simulink model "Zero_Perturb_MPPT_Live"  (R2025a)
settings: Solver=ode23t  StopTime=2  FixedStep=1e-6  MaxStep=2e-6
InitFcn:
  | if ~exist('PI_Preset','var'), PI_Preset = 'sun'; end
  | switch PI_Preset
  |   case 'bench'  % doc constants, indoor-lamp bench (3-5% duty)
  |     PI_Kp=1.2; PI_Ki=0.5; PI_Vdb=0.04; PI_Umax=600; PI_Slew=1; PI_Duty0=150;
  |   otherwise       % full-sun / cloud transient (retuned, see report)
  |     PI_Kp=100; PI_Ki=2500; PI_Vdb=0.04; PI_Umax=3900; PI_Slew=1000; PI_Duty0=2500;
  | end
  | PI_Ts = 0.05;
StartFcn:
  | fprintf('\n[SIMULINK LIVE] Simulation Started. Streaming to http://localhost:3000...\n');
StopFcn:
  | fprintf('\n[SIMULINK LIVE] Simulation Stopped.\n');
libraries: nesl_utility x6, fl_lib x5, ee_lib x3, simulink x1
(part 1 of 2)
settings Model: Creator=admin  LastModifiedBy=saisi
settings SolverCC: ZeroCrossAlgorithm=Adaptive
settings DebuggingCC: AlgebraicLoopMsg=none

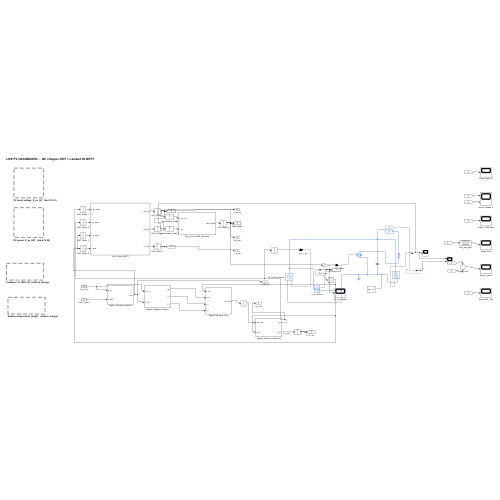
[thumbnail: Simulink's stored preview of the top-level diagram]
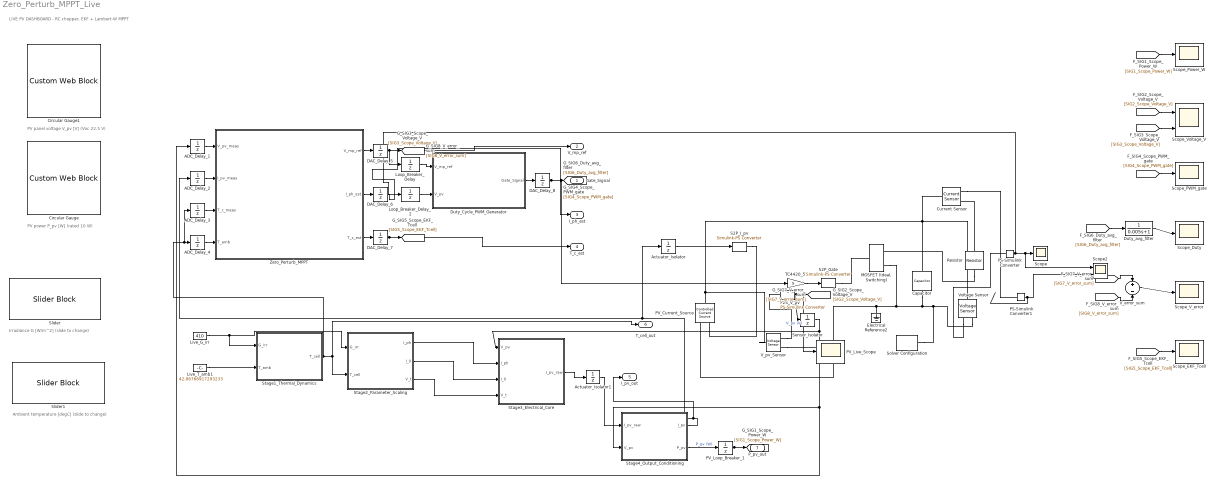
== system Zero_Perturb_MPPT_Live ==
  note: LIVE PV DASHBOARD - RC chopper, EKF + Lambert-W MPPT
  note: PV panel voltage V_pv [V] (Voc 22.5 V)
  note: PV power P_pv [W] (rated 10 W)
  note: Irradiance G [W/m^2] (slide to change)
  note: Ambient temperature [degC] (slide to change)
  ADC_Delay_{1..4} (4 alike) : UnitDelay  SampleTime=-1
  Actuator_Isolator : UnitDelay  SampleTime=-1
  Actuator_Isolator1 : UnitDelay  SampleTime=-1
  Capacitor : ee_lib/Passive/Capacitor  cap_option=ee.enum.passive.capacitor.capOption.const  c=470e-6 F  Cvec=[1e-05, 1e-06] F  Vvec=[0, 10] V  CV_table_symmetry=ee.enum.passive.capacitor.tableSymmetry.yes  f_vec=[1, 10] kHz  DFext_vec=[.8, 1.2]  enable_C_tol=ee.enum.toleranceApplication.none  averaging_period=0 s  C_tol=5  tol_distribution=ee.enum.toleranceDistribution.uniform  nSigma=4  r=0 Ohm  g=0 1/Ohm  enable_operating_limits=ee.enum.enable.no  operating_limit_action=ee.enum.passive.reportOpLim.warn  max_working_voltage_range=[-25, 25] V  power_rating=1 W  maxTemperature=85 degC  thermalEnable=false  thermalMass=1 J/K  i_specify=off  i_priority=None  i=0 A  i_nominal_specify=off  i_nominal_value=1  i_nominal_unit=A  v_specify=off  v_priority=None  v=0 V  v_nominal_specify=off  v_nominal_value=1  v_nominal_unit=V  vc_specify=off  vc_priority=High  vc=0 V  vc_nominal_specify=off  vc_nominal_value=1  vc_nominal_unit=V  T_specify=off  T_priority=None  T=298.15 K  T_nominal_specify=off  T_nominal_value=1  T_nominal_unit=K
  Circular Gauge : CustomWebBlock  ShowInitialText=on  Configuration="{\"components\":[{\"name\":\"CircularScaleComponent\",\"settings\":{\"bounds\":{\"max\":15,\"min\":0,\"tickInterval\":\"auto\"},\"direction\":\"cw\",\"flipLimits\":0,\"innerRadius\":0.75,\"internalTickHeightScaleFactor\":1,\"labelColor\":[255,255,200],\"labelFont\":{\"font\":\"Arial\",\"fontSize\":12},\"labelRadius\":0.528,\"labelTransparency\":1,\"minorTickHeightScaleFactor\":0.2,\"needleImage\":{\"size\":[200,50],\"src\":\"data:image\\/svg+xml;base64,PD94bWwgdmVyc2lvbj0iMS4wIiBlbmNvZGluZz0idXRmLTgiPz4KPCEtLSBHZW5lcmF0b3I6IEFkb2JlIElsbHVzdHJhdG9yIDI0LjEuMiwgU1ZHIEV4cG9ydCBQbHVnLUluIC4gU1ZHIFZlcnNpb246IDYuMDAgQnVpbGQgMCkgIC0tPgo8c3ZnIHZlcnNpb249IjEuMSIgaWQ9IkxheWVyXzEiIHhtbG5zPSJodHRwOi8vd3d3LnczLm9yZy8yMDAwL3N2ZyIgeG1sbnM6eGxpbms9Imh0dHA6Ly93d3cudzMub3JnLzE5OTkveGxpbmsiIHg9IjBweCIgeT0iMHB4IgoJIHZpZXdCb3g9IjAgMCAyMDAgNTAiIHN0eWxlPSJlbmFibGUtYmFja2dyb3VuZDpuZXcgMCAwIDIwMCA1MDsiIHhtbDpzcGFjZT0icHJlc2VydmUiPgo8c3R5bGUgdHlwZT0idGV4dC9jc3MiPgoJLnN0MHtmaWxsOiNFQzIxMjc7fQo8L3N0eWxlPgo8cGF0aCBjbGFzcz0ic3QwIiBkPSJNMTYyLjgsMTMuN0MxNjksNC40LDE4MS43LDEuOSwxOTEsOC4xczExLjgsMTguOSw1LjYsMjguMnMtMTguOSwxMS44LTI4LjIsNS42bDAsMAoJQzE1OS4xLDM1LjYsMTU2LjYsMjMsMTYyLjgsMTMuN0wxNjIuOCwxMy43eiBNMTY1LjgsMTUuOGMtNS4xLDcuNi0zLjEsMTcuOSw0LjYsMjNjNy42LDUuMSwxNy45LDMuMSwyMy00LjYKCWM1LjEtNy42LDMuMS0xNy45LTQuNi0yM2wwLDBDMTgxLjIsNi4yLDE3MC45LDguMiwxNjUuOCwxNS44eiIvPgo8cGF0aCBjbGFzcz0ic3QwIiBkPSJNMC40LDI1Ljl2LTMuM2wxNTktMi41Yy0wLjcsMi42LTAuNyw1LjIsMCw3LjhMMC40LDI1Ljl6Ii8+CjxjaXJjbGUgY2xhc3M9InN0MCIgY3g9IjE3OS42IiBjeT0iMjQiIHI9IjAuNyIvPgo8L3N2Zz4K\"},\"needleOffset\":[0.18464878250906522,0],\"needleOrientation\":-45,\"needleRotation\":180,\"needleSize\":{\"height\":0.11741692305346914,\"width\":0.46108337545091255},\"outerRadius\":0.9,\"position\":[0.05,0.05,0.9,0.9],\"referencePoint\":\"auto\",\"scaleAngle\":270,\"scaleAngleOffset\":135,\"scaleColors\":[],\"scaleColorsSize\":0.2,\"scaleDirection\":\"CW\",\"scalePosition\":[0,0,1,1],\"showLabels\":1,\"showMinorTicks\":1,\"showSpanLine\":1,\"showTicks\":1,\"tickColor\":[252,252,197],\"tickTransparency\":1,\"valueBarColor\":[0,114,189],\"valueBarPosition\":[0,0,1,1],\"valueBarSize\":0.2,\"valueBarTransparency\":1}},{\"name\":\"BackgroundImageComponent\",\"settings\":{\"image\":{\"size\":[500,500],\"src\":\"data:image\\/svg+xml;base64,PD94bWwgdmVyc2lvbj0iMS4wIiBlbmNvZGluZz0iVVRGLTgiIHN0YW5kYWxvbmU9Im5vIj8+CjxzdmcKICAgeG1sbnM6ZGM9Imh0dHA6Ly9wdXJsLm9yZy9kYy9lbGVtZW50cy8xLjEvIgogICB4bWxuczpjYz0iaHR0cDovL2NyZWF0aXZlY29tbW9ucy5vcmcvbnMjIgogICB4bWxuczpyZGY9Imh0dHA6Ly93d3cudzMub3JnLzE5OTkvMDIvMjItcmRmLXN5bnRheC1ucyMiCiAgIHhtbG5zOnN2Zz0iaHR0cDovL3d3dy53My5vcmcvMjAwMC9zdmciCiAgIHhtbG5zPSJodHRwOi8vd3d3LnczLm9yZy8yMDAwL3N2ZyIKICAgeG1sbnM6 ...(+9964 chars)\"},\"position\":[0,0,1,1],\"scaleMode\":\"0\"}},{\"name\":\"ForegroundImageComponent\",\"settings\":{\"image\":{\"size\":[0,0],\"src\":\"default\",\"srcOrientation\":[]},\"isForeground\":1,\"position\":[0,0,1,1],\"scaleMode\":\"0\"}}],\"derived\":{\"blockParameters\":{\"ForegroundColor\":[0.9882352941176471,0.9882352941176471,0.7725490196078432],\"Limits\":{\"Max\":15,\"Min\":0,\"Ticks\":\"auto\"},\"ScaleColors\":[],\"ScaleDirection\":\"Clockwise\",\"ScaleMax\":15,\"ScaleMin\":0,\"TickInterval\":\"auto\",\"fixedAspectRatio\":\"on\"}},\"settings\":{\"BindingType\":\"signal\",\"aspectRatio\":1.032258064516129,\"backgroundColor\":[0,0,0,\"1\"],\"backgroundOffset\":1,\"backgroundOpacity\":1,\"direction\":\"cw\",\"fixedAspectRatio\":\"on\",\"flipLimits\":0,\"orientation\":\"horizontal\",\"showBackgroundColor\":false,\"value\":0,\"version\":\"R2023a\"},\"type\":\"CircularGauge\"}"
  Circular Gauge1 : CustomWebBlock  ShowInitialText=on  Configuration="{\"components\":[{\"name\":\"CircularScaleComponent\",\"settings\":{\"bounds\":{\"max\":25,\"min\":0,\"tickInterval\":\"auto\"},\"direction\":\"cw\",\"flipLimits\":0,\"innerRadius\":0.75,\"internalTickHeightScaleFactor\":1,\"labelColor\":[255,255,200],\"labelFont\":{\"font\":\"Arial\",\"fontSize\":12},\"labelRadius\":0.528,\"labelTransparency\":1,\"minorTickHeightScaleFactor\":0.2,\"needleImage\":{\"size\":[200,50],\"src\":\"data:image\\/svg+xml;base64,PD94bWwgdmVyc2lvbj0iMS4wIiBlbmNvZGluZz0idXRmLTgiPz4KPCEtLSBHZW5lcmF0b3I6IEFkb2JlIElsbHVzdHJhdG9yIDI0LjEuMiwgU1ZHIEV4cG9ydCBQbHVnLUluIC4gU1ZHIFZlcnNpb246IDYuMDAgQnVpbGQgMCkgIC0tPgo8c3ZnIHZlcnNpb249IjEuMSIgaWQ9IkxheWVyXzEiIHhtbG5zPSJodHRwOi8vd3d3LnczLm9yZy8yMDAwL3N2ZyIgeG1sbnM6eGxpbms9Imh0dHA6Ly93d3cudzMub3JnLzE5OTkveGxpbmsiIHg9IjBweCIgeT0iMHB4IgoJIHZpZXdCb3g9IjAgMCAyMDAgNTAiIHN0eWxlPSJlbmFibGUtYmFja2dyb3VuZDpuZXcgMCAwIDIwMCA1MDsiIHhtbDpzcGFjZT0icHJlc2VydmUiPgo8c3R5bGUgdHlwZT0idGV4dC9jc3MiPgoJLnN0MHtmaWxsOiNFQzIxMjc7fQo8L3N0eWxlPgo8cGF0aCBjbGFzcz0ic3QwIiBkPSJNMTYyLjgsMTMuN0MxNjksNC40LDE4MS43LDEuOSwxOTEsOC4xczExLjgsMTguOSw1LjYsMjguMnMtMTguOSwxMS44LTI4LjIsNS42bDAsMAoJQzE1OS4xLDM1LjYsMTU2LjYsMjMsMTYyLjgsMTMuN0wxNjIuOCwxMy43eiBNMTY1LjgsMTUuOGMtNS4xLDcuNi0zLjEsMTcuOSw0LjYsMjNjNy42LDUuMSwxNy45LDMuMSwyMy00LjYKCWM1LjEtNy42LDMuMS0xNy45LTQuNi0yM2wwLDBDMTgxLjIsNi4yLDE3MC45LDguMiwxNjUuOCwxNS44eiIvPgo8cGF0aCBjbGFzcz0ic3QwIiBkPSJNMC40LDI1Ljl2LTMuM2wxNTktMi41Yy0wLjcsMi42LTAuNyw1LjIsMCw3LjhMMC40LDI1Ljl6Ii8+CjxjaXJjbGUgY2xhc3M9InN0MCIgY3g9IjE3OS42IiBjeT0iMjQiIHI9IjAuNyIvPgo8L3N2Zz4K\"},\"needleOffset\":[0.18464878250906522,0],\"needleOrientation\":-45,\"needleRotation\":180,\"needleSize\":{\"height\":0.11741692305346914,\"width\":0.46108337545091255},\"outerRadius\":0.9,\"position\":[0.05,0.05,0.9,0.9],\"referencePoint\":\"auto\",\"scaleAngle\":270,\"scaleAngleOffset\":135,\"scaleColors\":[],\"scaleColorsSize\":0.2,\"scaleDirection\":\"CW\",\"scalePosition\":[0,0,1,1],\"showLabels\":1,\"showMinorTicks\":1,\"showSpanLine\":1,\"showTicks\":1,\"tickColor\":[252,252,197],\"tickTransparency\":1,\"valueBarColor\":[0,114,189],\"valueBarPosition\":[0,0,1,1],\"valueBarSize\":0.2,\"valueBarTransparency\":1}},{\"name\":\"BackgroundImageComponent\",\"settings\":{\"image\":{\"size\":[500,500],\"src\":\"data:image\\/svg+xml;base64,PD94bWwgdmVyc2lvbj0iMS4wIiBlbmNvZGluZz0iVVRGLTgiIHN0YW5kYWxvbmU9Im5vIj8+CjxzdmcKICAgeG1sbnM6ZGM9Imh0dHA6Ly9wdXJsLm9yZy9kYy9lbGVtZW50cy8xLjEvIgogICB4bWxuczpjYz0iaHR0cDovL2NyZWF0aXZlY29tbW9ucy5vcmcvbnMjIgogICB4bWxuczpyZGY9Imh0dHA6Ly93d3cudzMub3JnLzE5OTkvMDIvMjItcmRmLXN5bnRheC1ucyMiCiAgIHhtbG5zOnN2Zz0iaHR0cDovL3d3dy53My5vcmcvMjAwMC9zdmciCiAgIHhtbG5zPSJodHRwOi8vd3d3LnczLm9yZy8yMDAwL3N2ZyIKICAgeG1sbnM6 ...(+9964 chars)\"},\"position\":[0,0,1,1],\"scaleMode\":\"0\"}},{\"name\":\"ForegroundImageComponent\",\"settings\":{\"image\":{\"size\":[0,0],\"src\":\"default\",\"srcOrientation\":[]},\"isForeground\":1,\"position\":[0,0,1,1],\"scaleMode\":\"0\"}}],\"derived\":{\"blockParameters\":{\"ForegroundColor\":[0.9882352941176471,0.9882352941176471,0.7725490196078432],\"Limits\":{\"Max\":25,\"Min\":0,\"Ticks\":\"auto\"},\"ScaleColors\":[],\"ScaleDirection\":\"Clockwise\",\"ScaleMax\":25,\"ScaleMin\":0,\"TickInterval\":\"auto\",\"fixedAspectRatio\":\"on\"}},\"settings\":{\"BindingType\":\"signal\",\"aspectRatio\":1.032258064516129,\"backgroundColor\":[0,0,0,\"1\"],\"backgroundOffset\":1,\"backgroundOpacity\":1,\"direction\":\"cw\",\"fixedAspectRatio\":\"on\",\"flipLimits\":0,\"orientation\":\"horizontal\",\"showBackgroundColor\":false,\"value\":0,\"version\":\"R2023a\"},\"type\":\"CircularGauge\"}"
  Current Sensor : fl_lib/Electrical/Electrical Sensors/Current Sensor
  DAC_Delay_{5..8} (4 alike) : UnitDelay  SampleTime=-1
  Duty_Cycle_PWM_Generator : Subsystem
  Duty_avg_filter : TransferFcn  Numerator=1  Denominator=[0.005 1]
  Electrical Reference2 : fl_lib/Electrical/Electrical Elements/Electrical Reference
  Live_G_irr : Constant  Value=410
  Live_T_amb1 : Constant  Value=42.06766917293233
  Loop_Breaker_Delay : UnitDelay  SampleTime=-1
  Loop_Breaker_Delay_2 : UnitDelay  SampleTime=-1
  "MOSFET (Ideal, Switching)" : ee_lib/Semiconductors & Converters/MOSFET (Ideal, Switching)  port_option=ee.enum.controlport.ps  Rds=0.022 Ohm  Goff=1e-6 1/Ohm  Vth=1.5 V  diode_param=ee.enum.semiconductors.protectionDiode.nodynamics  diode_Vf=0.8 V  diode_Ron=0.001 Ohm  diode_Goff=1e-5 1/Ohm  diode_C=50e-9 F  diode_iRM=-235 A  diode_iF=300 A  diode_idot=-50 A/us  diode_trr_param=ee.enum.converters.diodeReverseParam.trr_factor  diode_trr_factor=3  diode_trr=15 us  diode_Qrr=1500 s*uA  ids_specify=off  ids_priority=None  ids=0 A  ids_nominal_specify=off  ids_nominal_value=1  ids_nominal_unit=A  vds_specify=off  vds_priority=None  vds=0 V  vds_nominal_specify=off  vds_nominal_value=1  vds_nominal_unit=V  vgs_specify=off  vgs_priority=None  vgs=0 V  vgs_nominal_specify=off  vgs_nominal_value=1  vgs_nominal_unit=V  thermal_loss_option=ee.enum.converters.thermalLossOption.constantvalues  Von_data=[0, 1.8, 3.2, 6, 10, 16; 0, 2, 5.5, 9.5, 15, 25] V  Tj=[298.15, 448.15] K  Iout_data=[0, 20, 40, 60, 80, 100] A  tabulateWithVds=false  Eon_data=[0, 55.04, 124.57, 235.53, 362.12; 0, 71.25, 161.25, 304.88, 468.75] * 1e-6 J  Eoff_data=[0, 18, 30, 56.1, 76.5; 0, 22.5, 37.5, 70.13, 95.63] * 1e-6 J  Eon_data_3D=[zeros(2, 5, 3)] J  Eoff_data_3D=[zeros(2, 5, 3)] J  Tj_loss=[298.15, 448.15] K  Iout_data_loss=[0, 10, 20, 30, 40] A  Vds_loss=[0, 150, 300] V  Eon_scalar=22.86e-3 J  Eoff_scalar=17.14e-3 J  Voff=300 V  Iout_scalar=600 A  useCurrentFromPreviousCycle=false  useVoltageFromPreviousCycle=false  diodeModelType=ee.enum.converters.diodeModelType.pwl  diodeTableType=ee.enum.diode.tableType.IfMat  diode_ReverseIVType=ee.enum.diode.diodeReverseIV.constant  diode_IfMat=[.07, .12, .19, 1.75, 4.24, 7.32, 11.2; .16, .3, .72, 2.14, 4.02, 6.35, 9.12] A  diode_VfMat=[.9, 1.15, 1.25, 1.5, 1.75, 2.17, 2.6, 2.85; .58, .68, .75, 1.1, 1.38, 1.77, 2.27, 2.7] V  diode_TjVec=[25, 125] degC  diode_VfVec=[.5, .7, .9, 1.3, 1.7, 2.1, 2.5] V  diode_IfVec=[.1, .2, .5, 1, 2, 4, 7, 10] A  diode_IrMat=[1e-06, 2e-06, 5e-06, 1e-05, 2.5e-05, 5e-05, .0001; 2e-06, 5e-06, 1e-05, 4e-05, 8e-05, .0002, .0005] A  diode_VrMat=[10, 100, 200, 250, 300, 325, 350; 10, 70, 160, 220, 270, 300, 320] V  diode_VrVec=[10, 20, 40, 50, 70, 80, 100] V  diode_IrVec=[1e-06, 2e-06, 5e-06, 1e-05, 2e-05, 5e-05, .0001] A  diode_Vr=-600 V  diode_Ls=150 nH  diode_Erec=0.03 J  diode_rec_loss_model=ee.enum.diode.reverseRecoveryModelTabulateUpTo3D.fixed  diode_ErecVal=0 J  diode_scaleWithIandV=true  diode_ErecMat=zeros(2, 3) J  diodeErecMat3D=zeros(2, 3, 2) J  diode_TjrecVec=[298.15, 398.15] K  diode_IfrecVec=[.1, 1, 10] A  diodeVrecVec=[0, 100] V  diode_IrecVal=10 A  diode_VrecVal=10 V  diode_tFilter=1 / 1000 / 100 s  separateThermalPortForDiode=false  thermal_network_parameterization=ee.enum.thermalNetworkTopology.external  Rth=[.03, .2] K/W  Rth_Cauer=[.03, .1, .2] K/W  Rth_Foster=[.08, .14, .22, .16] K/W  thermal_mass_parameterization=ee.enum.thermalNetwork.timeconstant  thermal_mass=[3, 25] J/K  thermal_mass_Cauer=[3, 10, 25] J/K  thermal_mass_Foster=[.001, .005, .05, .5] J/K  thermal_time_constant=[.1, 5] s  thermal_time_constant_Cauer=[.1, 1, 5] s  thermal_time_constant_Foster=[7e-05, .0007, .01, .08] s  thermal_mass_initial_temperatures=[25, 25] degC  thermal_mass_initial_temperatures_Cauer=[25, 25, 25] degC  junction_thermal_mass=0.1 J/K  Tvec_initial_Foster=[25, 25, 25, 25] degC  RthDiode=[.03, .2] K/W  RthCauerDiode=[.03, .1, .2] K/W  RthFosterDiode=[.03, .2] K/W  thermalMassDiode=[3, 25] J/K  thermalMassCauerDiode=[3, 10, 25] J/K  thermalMassFosterDiode=[33, 50] J/K  thermalTauDiode=[.1, 5] s  thermalTauCauerDiode=[.1, 1, 5] s  thermalTauFosterDiode=[1, 10] s  thermalMassInitTempDiode=[25, 25] degC  thermalMassInitTempCauerDiode=[25, 25, 25] degC  junctionthermalMassDiode=0.1 J/K  TVecInitialFosterDiode=[25, 25, 25, 25] degC  no_thermal_network=ee.enum.enable.no  mosfet_junction_temperature_specify=off  mosfet_junction_temperature_priority=None  mosfet_junction_temperature=25 degC  mosfet_junction_temperature_nominal_specify=off  mosfet_junction_temperature_nominal_value=1  mosfet_junction_temperature_nominal_unit=degC  diode_junction_temperature_specify=off  diode_junction_temperature_priority=None  diode_junction_temperature=25 degC  diode_junction_temperature_nominal_specify=off  diode_junction_temperature_nominal_value=1  diode_junction_temperature_nominal_unit=degC  Qj_specify=off  Qj_priority=None  Qj=0 W  Qj_nominal_specify=off  Qj_nominal_value=1  Qj_nominal_unit=W  accumulatedSwitchingLosses_specify=off  accumulatedSwitchingLosses_priority=None  accumulatedSwitchingLosses=0 J
  P2S_V_pv : nesl_utility/PS-Simulink Converter  PhysicalDomain=network_engine_domain  SubClassName=ps_output  LeftPortType=input  RightPortType=output  PseudoPeriodic=off  Frequencies=[]  VectorFormat=inherit  Unit=inherit  AffineConversion=off
  PS-Simulink Converter : nesl_utility/PS-Simulink Converter  PhysicalDomain=network_engine_domain  SubClassName=ps_output  LeftPortType=input  RightPortType=output  PseudoPeriodic=off  Frequencies=[]  VectorFormat=inherit  Unit=inherit  AffineConversion=off
  PS-Simulink Converter1 : nesl_utility/PS-Simulink Converter  PhysicalDomain=network_engine_domain  SubClassName=ps_output  LeftPortType=input  RightPortType=output  PseudoPeriodic=off  Frequencies=[]  VectorFormat=inherit  Unit=inherit  AffineConversion=off
  PV_Current_Source : fl_lib/Electrical/Electrical Sources/Controlled Current Source
  PV_Live_Scope : Scope
      settings: ActiveDisplayYMinimum=-13.90968560609708  ActiveDisplayYMaximum=19.630172966597019
  PV_Loop_Breaker_1 : UnitDelay  SampleTime=-1
  Resistor : ee_lib/Passive/Resistor  R=23.5 Ohm  enable_R_tol=ee.enum.toleranceApplication.none  R_tol=5  tol_distribution=ee.enum.toleranceDistribution.uniform  nSigma=4  enable_operating_limits=ee.enum.enable.no  operating_limit_action=ee.enum.passive.reportOpLim.warn  power_rating=1 W  max_working_voltage=100 V  noise_mode=ee.enum.sources.noise.Disabled  Tdevice=25 degC  sample_time=1e-3 s  repeatability=ee.enum.ic.repeatability.notRepeatable  user_seed=0  auto_seed=2048266675  power_derating_T1=70 degC  power_derating_T2=155 degC  operating_temperature_range_vec=[-50, 150] degC  alpha=3.93e-3 1/K  Tmeas=25 degC  thermal_mass=100 J/K  temperature_specify=off  temperature_priority=High  temperature=298.15 K  temperature_nominal_specify=off  temperature_nominal_value=1  temperature_nominal_unit=K
  S2P_Gate : nesl_utility/Simulink-PS Converter  PhysicalDomain=network_engine_domain  SubClassName=ps_input  LeftPortType=input  RightPortType=output  PseudoPeriodic=off  Frequencies=[]  NoiseDistribution=none  NoiseParameters=[]  Unit=1  AffineConversion=off  FilteringAndDerivatives=zero  SimscapeFilterOrder=1  InputFilterTimeConstant=0.001  UdotUserProvided=0
  S2P_I_pv : nesl_utility/Simulink-PS Converter  PhysicalDomain=network_engine_domain  SubClassName=ps_input  LeftPortType=input  RightPortType=output  PseudoPeriodic=off  Frequencies=[]  NoiseDistribution=none  NoiseParameters=[]  Unit=1  AffineConversion=off  FilteringAndDerivatives=filter  SimscapeFilterOrder=1  InputFilterTimeConstant=0.001  UdotUserProvided=0
  Scope : Scope
      settings: ActiveDisplayYMinimum=13.007954548384831  ActiveDisplayYMaximum=31.502856897275876
  Scope2 : Scope  NumInputPorts=2
      settings: ActiveDisplayYMinimum=-25.731009602187875  ActiveDisplayYMaximum=24.316199823397437  DataLoggingVariableName=ScopeData2
  Scope_Duty : Scope
      settings: Title=Duty cycle (averaged PWM)
  Scope_EKF_Tcell : Scope
      settings: Title=EKF estimated cell temperature [degC]
  Scope_PWM_gate : Scope
      settings: TimeSpan=0.0005  Title=PWM gate signal (10 kHz, last 0.5 ms)
  Scope_Power_W : Scope
      settings: Title=PV power P_pv [W]
  Scope_V_error : Scope
      settings: Title=V_pv - V_mp_ref [V] (tracking error)
  Scope_Voltage_V : Scope  NumInputPorts=2
      settings: Title=V_pv (meas) and V_mp_ref (EKF target) [V]
  Sensor_Isolator : UnitDelay  SampleTime=-1
  Slider : SliderBlock  ScaleMin=50  ScaleMax=1200
  Slider1 : SliderBlock  ScaleMin=15  ScaleMax=65
  Solver Configuration : nesl_utility/Solver Configuration  PhysicalDomain=network_engine_domain  SubClassName=solver  LeftPortType=input  RightPortType=generic  Tones=[]  Harmonics=[]  SimulateNoise=off  Profile=off  UseLocalSampling=off  EnableSwitchedLinearOptims=on  FrequencyDomain=off  UseCCode=off  RelTol=0.001  AbsTol=0.001  MinStep=1e-09  ToWorkspace=off  RevertToSquareIcSolve=off  NumHomotopyIterations=100  PhasorMode=off  PhasorModeNumHarmonics=1  ConsistencySolver=NEWTON_XTOL_AFTER_FTOL  CanonicalOrdering=UNORDERED  OptimizeIntermediates=UNOPTIMIZED  IndexReductionMethod=DerivativeReplacement  DoDC=off  ResidualTolerance=1e-09  ConsistencyTolSource=GLOBAL  ConsistencyAbsTol=0.001  ConsistencyRelTol=0.001  ConsistencyTolFactor=0.001  UseLocalSolver=on  LocalSolverChoice=NE_BACKWARD_EULER_ADVANCER  ResolveIndetEquations=on  FunctionEvalNumThread=1  LocalSolverSampleTime=0.000001  DoFixedCost=off  MaxNonlinIter=3  MaxModeIter=2  ComputeImpulses=off  ImpulseIterations=2  LinearAlgebra=auto  LinearAlgebraNumThread=0  EquationFormulation=NE_TIME_EF  DelaysMemoryBudget=1024  AutomaticFiltering=on  FilteringTimeConstant=0.001  PartitionStorageMethod=AS_NEEDED  PartitionMemoryBudget=1024  PartitionMethod=ROBUST  MultibodyUseLocalSolver=off  MultibodyLocalSolverChoice=ODE1  MultibodyLocalSolverSampleTime=0.001
  Stage1_Thermal_Dynamics : Subsystem
  Stage2_Parameter_Scaling : Subsystem
  Stage3_Electrical_Core : Subsystem
  Stage4_Output_Conditioning : Subsystem
  TC4420_5V : Gain  Gain=5
  V_error_sum : Sum  Inputs=+-
  V_pv_Sensor : fl_lib/Electrical/Electrical Sensors/Voltage Sensor
  Voltage Sensor : fl_lib/Electrical/Electrical Sensors/Voltage Sensor
  Zero_Perturb_MPPT : Subsystem
  Gate_Signal : Outport
  V_mp_ref : Outport  Port=2
  I_ph_est : Outport  Port=3
  T_c_est : Outport  Port=4
  I_pv_out : Outport  Port=5
  T_cell_out : Outport  Port=6
  P_pv_out : Outport  Port=7
  wires:
  PS-Simulink Converter/1 -> Scope2/1, Scope/1, Loop_Breaker_Delay_2/1
  PS-Simulink Converter1/1 -> Scope2/2
  Stage4_Output_Conditioning/1(I_pv) -> ADC_Delay_2/1, Actuator_Isolator/1, I_pv_out/1
  Stage1_Thermal_Dynamics/1(T_cell) -> ADC_Delay_3/1, ADC_Delay_4/1, Stage2_Parameter_Scaling/2(T_cell), T_cell_out/1
  Stage2_Parameter_Scaling/3(V_t) -> Stage3_Electrical_Core/4(V_t)
  Stage2_Parameter_Scaling/1(I_ph) -> Stage3_Electrical_Core/2(I_ph)
  Stage2_Parameter_Scaling/2(I_0) -> Stage3_Electrical_Core/3(I_0)
  Live_G_irr/1 -> Stage1_Thermal_Dynamics/1(G_irr), Stage2_Parameter_Scaling/1(G_irr)
  Live_T_amb1/1 -> Stage1_Thermal_Dynamics/2(T_amb)
  Loop_Breaker_Delay/1 -> Duty_Cycle_PWM_Generator/1(V_mp_ref)
  Loop_Breaker_Delay_2/1 -> Duty_Cycle_PWM_Generator/2(V_pv)
  ADC_Delay_1/1 -> Zero_Perturb_MPPT/1(V_pv_meas)
  ADC_Delay_2/1 -> Zero_Perturb_MPPT/2(I_pv_meas)
  ADC_Delay_3/1 -> Zero_Perturb_MPPT/3(T_c_meas)
  ADC_Delay_4/1 -> Zero_Perturb_MPPT/4(T_amb)
  Zero_Perturb_MPPT/1(V_mp_ref) -> DAC_Delay_5/1
  DAC_Delay_5/1 -> V_mp_ref/1, Loop_Breaker_Delay/1, [SIG3_Scope_Voltage_V], [SIG8_V_error_sum]
  Zero_Perturb_MPPT/2(I_ph_est) -> DAC_Delay_6/1
  DAC_Delay_6/1 -> I_ph_est/1
  Zero_Perturb_MPPT/3(T_c_est) -> DAC_Delay_7/1
  DAC_Delay_7/1 -> T_c_est/1, [SIG5_Scope_EKF_Tcell]
  Duty_Cycle_PWM_Generator/1(Gate_Signal) -> DAC_Delay_8/1
  DAC_Delay_8/1 -> Gate_Signal/1, TC4420_5V/1, [SIG4_Scope_PWM_gate], [SIG6_Duty_avg_filter]
  Stage4_Output_Conditioning/2(P_pv) -> PV_Loop_Breaker_1/1  "P_pv (W)"
  PV_Loop_Breaker_1/1 -> P_pv_out/1, [SIG1_Scope_Power_W]
  P2S_V_pv/1 -> Sensor_Isolator/1, PV_Live_Scope/1, [SIG2_Scope_Voltage_V], [SIG7_V_error_sum]  "V_pv (V)"
  Sensor_Isolator/1 -> ADC_Delay_1/1, Stage4_Output_Conditioning/2(V_pv), Stage3_Electrical_Core/1(V_pv)
  Actuator_Isolator/1 -> S2P_I_pv/1
  Stage3_Electrical_Core/1(I_pv_raw) -> Actuator_Isolator1/1
  Actuator_Isolator1/1 -> Stage4_Output_Conditioning/1(I_pv_raw)
  TC4420_5V/1 -> S2P_Gate/1
  ? -> ?
  Duty_avg_filter/1 -> Scope_Duty/1
  V_error_sum/1 -> Scope_V_error/1
  [SIG1_Scope_Power_W] -> Scope_Power_W/1
  [SIG2_Scope_Voltage_V] -> Scope_Voltage_V/1
  [SIG3_Scope_Voltage_V] -> Scope_Voltage_V/2
  [SIG4_Scope_PWM_gate] -> Scope_PWM_gate/1
  [SIG5_Scope_EKF_Tcell] -> Scope_EKF_Tcell/1
  [SIG6_Duty_avg_filter] -> Duty_avg_filter/1
  [SIG7_V_error_sum] -> V_error_sum/1
  [SIG8_V_error_sum] -> V_error_sum/2
  connections:
  Resistor/LConn1 -- Current Sensor/RConn2
  Current Sensor/RConn1 -- PS-Simulink Converter1/LConn1
  Voltage Sensor/RConn1 -- PS-Simulink Converter/LConn1
  S2P_Gate/RConn1 -- "MOSFET (Ideal, Switching)"/LConn1
  S2P_I_pv/RConn1 -- PV_Current_Source/RConn1
  V_pv_Sensor/RConn1 -- P2S_V_pv/LConn1
  Electrical Reference2/LConn1 -- Solver Configuration/RConn1 -- Voltage Sensor/RConn2 -- Capacitor/RConn1 -- "MOSFET (Ideal, Switching)"/RConn2 -- PV_Current_Source/RConn2 -- V_pv_Sensor/RConn2
  V_pv_Sensor/LConn1 -- PV_Current_Source/LConn1 -- Capacitor/LConn1 -- Voltage Sensor/LConn1 -- Current Sensor/LConn1
  Resistor/RConn1 -- "MOSFET (Ideal, Switching)"/RConn1

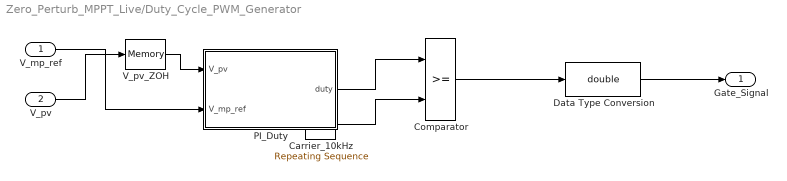
== system Zero_Perturb_MPPT_Live/Duty_Cycle_PWM_Generator ==
  V_mp_ref : Inport
  V_pv : Inport  Port=2
  Carrier_10kHz : simulink/Sources/Repeating Sequence  rep_seq_t=[0 1e-4]  rep_seq_y=[0 1]
  Comparator : RelationalOperator  OutDataTypeStr=boolean  RndMeth=Simplest  InputSameDT=off
  Data Type Conversion : DataTypeConversion  OutDataTypeStr=double  SaturateOnIntegerOverflow=off  RndMeth=Floor
  PI_Duty : MATLAB Function  TreatAsAtomicUnit=on
  V_pv_ZOH : Memory  InitialCondition=19
  Gate_Signal : Outport
  wires:
  V_pv/1 -> V_pv_ZOH/1
  V_pv_ZOH/1 -> PI_Duty/1(V_pv)
  V_mp_ref/1 -> PI_Duty/2(V_mp_ref)
  PI_Duty/1(duty) -> Comparator/1
  Carrier_10kHz/1 -> Comparator/2
  Comparator/1 -> Data Type Conversion/1
  Data Type Conversion/1 -> Gate_Signal/1

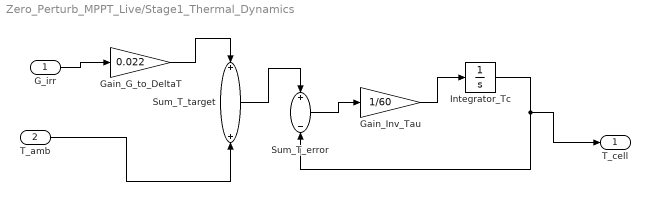
== system Zero_Perturb_MPPT_Live/Stage1_Thermal_Dynamics ==
  G_irr : Inport
  T_amb : Inport  Port=2
  Gain_G_to_DeltaT : Gain  Gain=0.022
  Gain_Inv_Tau : Gain  Gain=1/60
  Integrator_Tc : Integrator  InitialCondition=28.0
  Sum_T_error : Sum  Inputs=+-
  Sum_T_target : Sum
  T_cell : Outport
  wires:
  G_irr/1 -> Gain_G_to_DeltaT/1
  Gain_G_to_DeltaT/1 -> Sum_T_target/1
  T_amb/1 -> Sum_T_target/2
  Sum_T_target/1 -> Sum_T_error/1
  Sum_T_error/1 -> Gain_Inv_Tau/1
  Gain_Inv_Tau/1 -> Integrator_Tc/1
  Integrator_Tc/1 -> Sum_T_error/2, T_cell/1

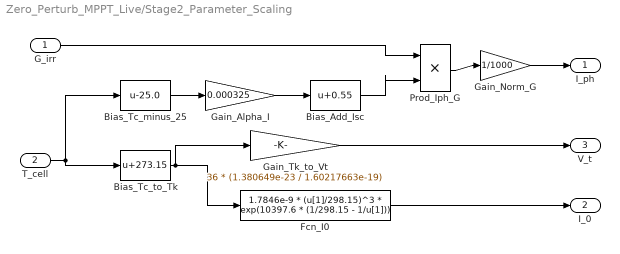
== system Zero_Perturb_MPPT_Live/Stage2_Parameter_Scaling ==
  G_irr : Inport
  T_cell : Inport  Port=2
  Bias_Add_Isc : Bias  Bias=0.55  SaturateOnIntegerOverflow=off
  Bias_Tc_minus_25 : Bias  Bias=-25.0  SaturateOnIntegerOverflow=off
  Bias_Tc_to_Tk : Bias  Bias=273.15  SaturateOnIntegerOverflow=off
  Fcn_I0 : Fcn  Expr=1.7846e-9 * (u[1]/298.15)^3 * exp(10397.6 * (1/298.15 - 1/u[1]))
  Gain_Alpha_I : Gain  Gain=0.000325
  Gain_Norm_G : Gain  Gain=1/1000
  Gain_Tk_to_Vt : Gain  Gain=36 * (1.380649e-23 / 1.60217663e-19)
  Prod_Iph_G : Product  Inputs=**
  I_ph : Outport
  I_0 : Outport  Port=2
  V_t : Outport  Port=3
  wires:
  T_cell/1 -> Bias_Tc_to_Tk/1, Bias_Tc_minus_25/1
  Bias_Tc_to_Tk/1 -> Gain_Tk_to_Vt/1, Fcn_I0/1
  Bias_Tc_minus_25/1 -> Gain_Alpha_I/1
  Gain_Alpha_I/1 -> Bias_Add_Isc/1
  G_irr/1 -> Prod_Iph_G/1
  Bias_Add_Isc/1 -> Prod_Iph_G/2
  Prod_Iph_G/1 -> Gain_Norm_G/1
  Gain_Norm_G/1 -> I_ph/1
  Fcn_I0/1 -> I_0/1
  Gain_Tk_to_Vt/1 -> V_t/1

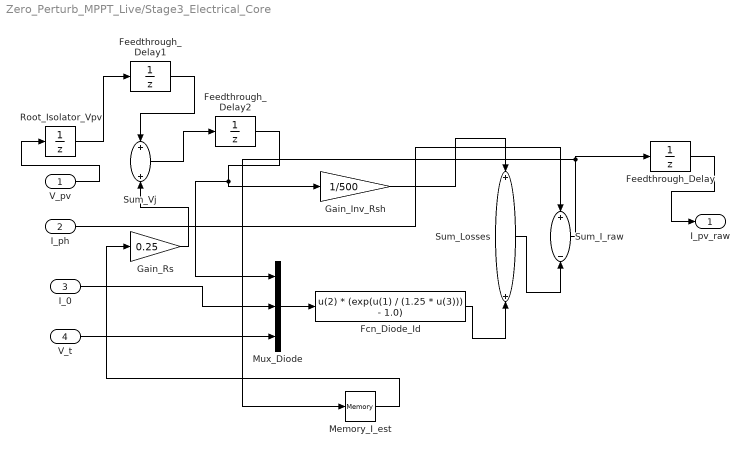
== system Zero_Perturb_MPPT_Live/Stage3_Electrical_Core ==
  V_pv : Inport
  I_ph : Inport  Port=2
  I_0 : Inport  Port=3
  V_t : Inport  Port=4
  Fcn_Diode_Id : Fcn  Expr=u(2) * (exp(u(1) / (1.25 * u(3))) - 1.0)
  Feedthrough_Delay : UnitDelay  SampleTime=-1
  Feedthrough_Delay1 : UnitDelay  SampleTime=-1
  Feedthrough_Delay2 : UnitDelay  SampleTime=-1
  Gain_Inv_Rsh : Gain  Gain=1/500
  Gain_Rs : Gain  Gain=0.25
  Memory_I_est : Memory  InitialCondition=0.55
  Mux_Diode : Mux  Inputs=3
  Root_Isolator_Vpv : UnitDelay  SampleTime=-1
  Sum_I_raw : Sum  Inputs=+-
  Sum_Losses : Sum
  Sum_Vj : Sum
  I_pv_raw : Outport
  wires:
  Gain_Rs/1 -> Sum_Vj/2
  Feedthrough_Delay2/1 -> Mux_Diode/1, Gain_Inv_Rsh/1
  Gain_Inv_Rsh/1 -> Sum_Losses/1
  I_0/1 -> Mux_Diode/2
  V_t/1 -> Mux_Diode/3
  Mux_Diode/1 -> Fcn_Diode_Id/1
  Fcn_Diode_Id/1 -> Sum_Losses/2
  I_ph/1 -> Sum_I_raw/1
  Sum_Losses/1 -> Sum_I_raw/2
  Sum_I_raw/1 -> Memory_I_est/1, Feedthrough_Delay/1
  Memory_I_est/1 -> Gain_Rs/1
  Feedthrough_Delay/1 -> I_pv_raw/1
  Feedthrough_Delay1/1 -> Sum_Vj/1
  Sum_Vj/1 -> Feedthrough_Delay2/1
  V_pv/1 -> Root_Isolator_Vpv/1
  Root_Isolator_Vpv/1 -> Feedthrough_Delay1/1

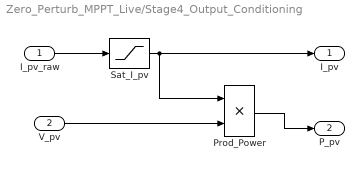
== system Zero_Perturb_MPPT_Live/Stage4_Output_Conditioning ==
  I_pv_raw : Inport
  V_pv : Inport  Port=2
  Prod_Power : Product  Inputs=**
  Sat_I_pv : Saturate  UpperLimit=0.60  LowerLimit=0.0  ZeroCross=off
  I_pv : Outport
  P_pv : Outport  Port=2
  wires:
  I_pv_raw/1 -> Sat_I_pv/1
  Sat_I_pv/1 -> I_pv/1, Prod_Power/1
  V_pv/1 -> Prod_Power/2
  Prod_Power/1 -> P_pv/1

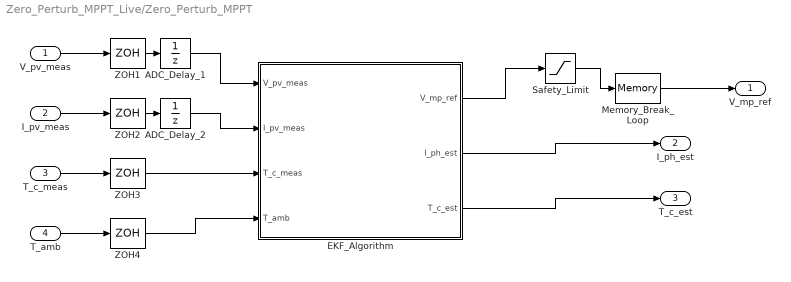
== system Zero_Perturb_MPPT_Live/Zero_Perturb_MPPT ==
  V_pv_meas : Inport
  I_pv_meas : Inport  Port=2
  T_c_meas : Inport  Port=3
  T_amb : Inport  Port=4
  ADC_Delay_1 : UnitDelay  SampleTime=0.05
  ADC_Delay_2 : UnitDelay  SampleTime=0.05
  EKF_Algorithm : MATLAB Function  TreatAsAtomicUnit=on
  Memory_Break_Loop : Memory  InitialCondition=19  InheritSampleTime=on
  Safety_Limit : Saturate  UpperLimit=22.5  LowerLimit=5.0
  ZOH{1..4} (4 alike) : ZeroOrderHold  SampleTime=0.05
  V_mp_ref : Outport
  I_ph_est : Outport  Port=2
  T_c_est : Outport  Port=3
  wires:
  V_pv_meas/1 -> ZOH1/1
  I_pv_meas/1 -> ZOH2/1
  T_c_meas/1 -> ZOH3/1
  T_amb/1 -> ZOH4/1
  ZOH3/1 -> EKF_Algorithm/3(T_c_meas)
  ZOH4/1 -> EKF_Algorithm/4(T_amb)
  EKF_Algorithm/1(V_mp_ref) -> Safety_Limit/1
  EKF_Algorithm/2(I_ph_est) -> I_ph_est/1
  EKF_Algorithm/3(T_c_est) -> T_c_est/1
  Safety_Limit/1 -> Memory_Break_Loop/1
  Memory_Break_Loop/1 -> V_mp_ref/1
  ZOH1/1 -> ADC_Delay_1/1
  ADC_Delay_1/1 -> EKF_Algorithm/1(V_pv_meas)
  ZOH2/1 -> ADC_Delay_2/1
  ADC_Delay_2/1 -> EKF_Algorithm/2(I_pv_meas)

== matlab function Zero_Perturb_MPPT_Live/Duty_Cycle_PWM_Generator/PI_Duty ==
  settings: updateMethod=DISCRETE  sampleTime=0.05
  data: V_pv input; duty output; V_mp_ref input; PI_Kp parameter; PI_Ki parameter; PI_Vdb parameter; PI_Ts parameter; PI_Umax parameter; PI_Slew parameter; PI_Duty0 parameter
function duty = PI_Duty(V_pv, V_mp_ref, PI_Kp, PI_Ki, PI_Vdb, PI_Ts, PI_Umax, PI_Slew, PI_Duty0)
    % Discrete Tustin bilinear PI (CIRCUIT_AND_LOGIC_DESCRIPTION s5.3), output = PWM duty (0..1)
    % e = V_pv - V_mp_ref : e>0 -> raise duty (load pulls the panel voltage down)
    persistent e_prev u_pi active
    if isempty(active)
        e_prev = 0.0;
        u_pi   = PI_Duty0;
        active = PI_Duty0;
    end
    e = V_pv - V_mp_ref;
    if abs(e) > PI_Vdb                                   % anti-hunting deadband (frozen inside)
        u_pi = u_pi + PI_Kp * (e - e_prev) + PI_Ki * (PI_Ts / 2.0) * (e + e_prev);
    end
    e_prev = e;
    u_pi   = min(max(u_pi, 0.0), PI_Umax);               % anti-windup clamp [0, Umax] counts
    active = active + min(max(u_pi - active, -PI_Slew), PI_Slew);   % slew limit counts/tick
    duty   = round(active) / 4095.0;                     % 12-bit LEDC resolution
end
